simulink model "plasma_load"  (R2026a)
settings: Solver=FixedStepDiscrete  StartTime=0  StopTime=30  FixedStep=1e-5
libraries: ee_lib x17, nesl_utility x13, fl_lib x9
settings Model: ModifiedByFormat=GKC3-Simulink contributors  Creator=GKC3-Simulink contributors  LastModifiedBy=GKC3-Simulink contributors
settings DataIOCC: FinalStateName=xHalf  InitialState=xHalf

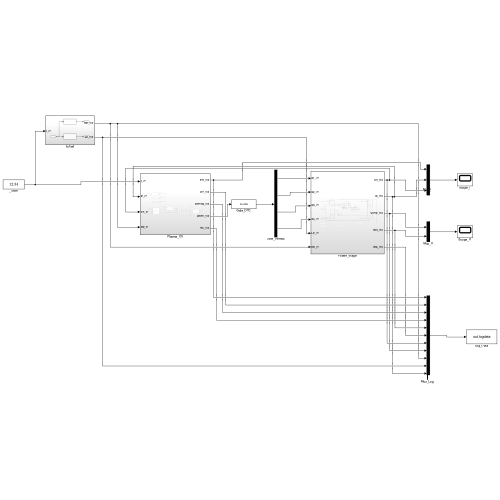
[thumbnail: Simulink's stored preview of the top-level diagram]
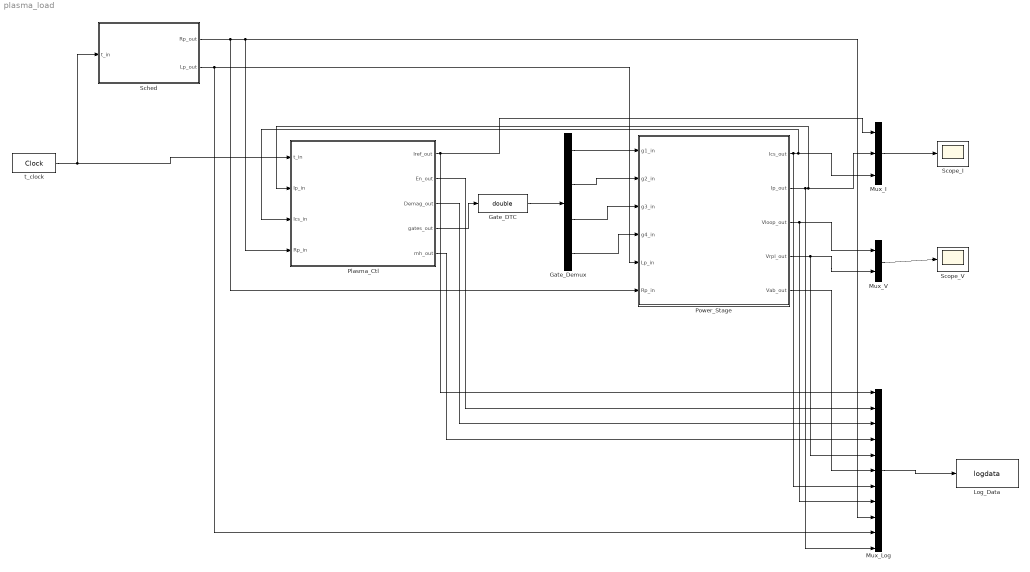
== system plasma_load ==
  Gate_DTC : DataTypeConversion  OutDataTypeStr=double  SaturateOnIntegerOverflow=off  RndMeth=Floor
  Gate_Demux : Demux
  Log_Data : ToWorkspace  VariableName=logdata  SaveFormat=Timeseries  SampleTime=1e-5
  Mux_I : Mux  Inputs=3
  Mux_Log : Mux  Inputs=11
  Mux_V : Mux  Inputs=2
  Plasma_Ctl : Subsystem
  Power_Stage : Subsystem
  Sched : Subsystem
  Scope_I : Scope
  Scope_V : Scope
  t_clock : DigitalClock  SampleTime=1e-5
  wires:
  Plasma_Ctl/4(gates_out) -> Gate_DTC/1
  Gate_DTC/1 -> Gate_Demux/1
  Gate_Demux/1 -> Power_Stage/1(g1_in)
  Gate_Demux/2 -> Power_Stage/2(g2_in)
  Gate_Demux/3 -> Power_Stage/3(g3_in)
  Gate_Demux/4 -> Power_Stage/4(g4_in)
  Mux_V/1 -> Scope_V/1
  t_clock/1 -> Sched/1(t_in), Plasma_Ctl/1(t_in)
  Sched/1(Rp_out) -> Plasma_Ctl/4(Rp_in), Mux_Log/9, Power_Stage/6(Rp_in)
  Sched/2(Lp_out) -> Power_Stage/5(Lp_in), Mux_Log/10
  Power_Stage/1(Ics_out) -> Mux_I/3, Plasma_Ctl/3(Ics_in), Mux_Log/7
  Power_Stage/2(Ip_out) -> Mux_I/2, Plasma_Ctl/2(Ip_in), Mux_Log/11
  Plasma_Ctl/1(Iref_out) -> Mux_Log/1, Mux_I/1
  Power_Stage/3(Vloop_out) -> Mux_V/1, Mux_Log/8
  Power_Stage/4(Vrpl_out) -> Mux_V/2, Mux_Log/5
  Plasma_Ctl/2(En_out) -> Mux_Log/2
  Plasma_Ctl/3(Demag_out) -> Mux_Log/3
  Plasma_Ctl/5(mh_out) -> Mux_Log/4
  Power_Stage/5(Vab_out) -> Mux_Log/6
  Mux_Log/1 -> Log_Data/1
  Mux_I/1 -> Scope_I/1

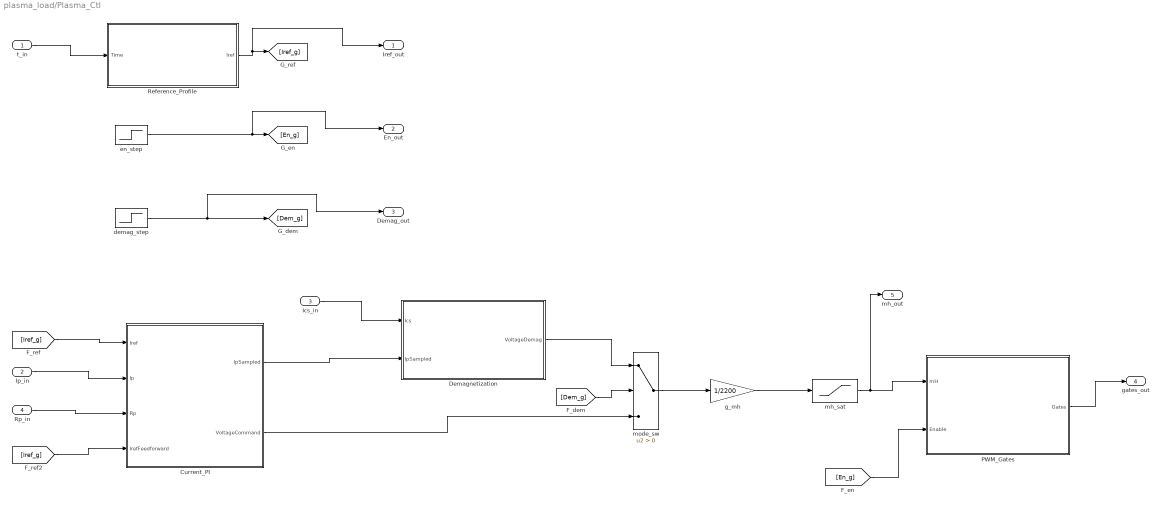
== system plasma_load/Plasma_Ctl ==
  t_in : Inport
  Ip_in : Inport  Port=2
  Ics_in : Inport  Port=3
  Rp_in : Inport  Port=4
  Current_PI : Subsystem
  Demagnetization : Subsystem
  PWM_Gates : Subsystem
  Reference_Profile : Subsystem
  demag_step : Step  Time=12.3  SampleTime=0
  en_step : Step  Time=0.6  SampleTime=0
  g_mh : Gain  Gain=1/2200
  mh_sat : Saturate  UpperLimit=0.95  LowerLimit=-0.95
  mode_sw : Switch  Criteria=u2 > Threshold  SaturateOnIntegerOverflow=off  InputSameDT=off
  Iref_out : Outport
  En_out : Outport  Port=2
  Demag_out : Outport  Port=3
  gates_out : Outport  Port=4
  mh_out : Outport  Port=5
  wires:
  mode_sw/1 -> g_mh/1
  [Dem_g] -> mode_sw/2
  demag_step/1 -> [Dem_g], Demag_out/1
  en_step/1 -> [En_g], En_out/1
  PWM_Gates/1(Gates) -> gates_out/1
  [En_g] -> PWM_Gates/2(Enable)
  Demagnetization/1(VoltageDemag) -> mode_sw/1
  Current_PI/1(IpSampled) -> Demagnetization/2(IpSampled)
  Ics_in/1 -> Demagnetization/1(Ics)
  Current_PI/2(VoltageCommand) -> mode_sw/3
  [Iref_g] -> Current_PI/4(IrefFeedforward)
  Rp_in/1 -> Current_PI/3(Rp)
  Ip_in/1 -> Current_PI/2(Ip)
  [Iref_g] -> Current_PI/1(Iref)
  t_in/1 -> Reference_Profile/1(Time)
  Reference_Profile/1(Iref) -> Iref_out/1, [Iref_g]
  g_mh/1 -> mh_sat/1
  mh_sat/1 -> PWM_Gates/1(mH), mh_out/1

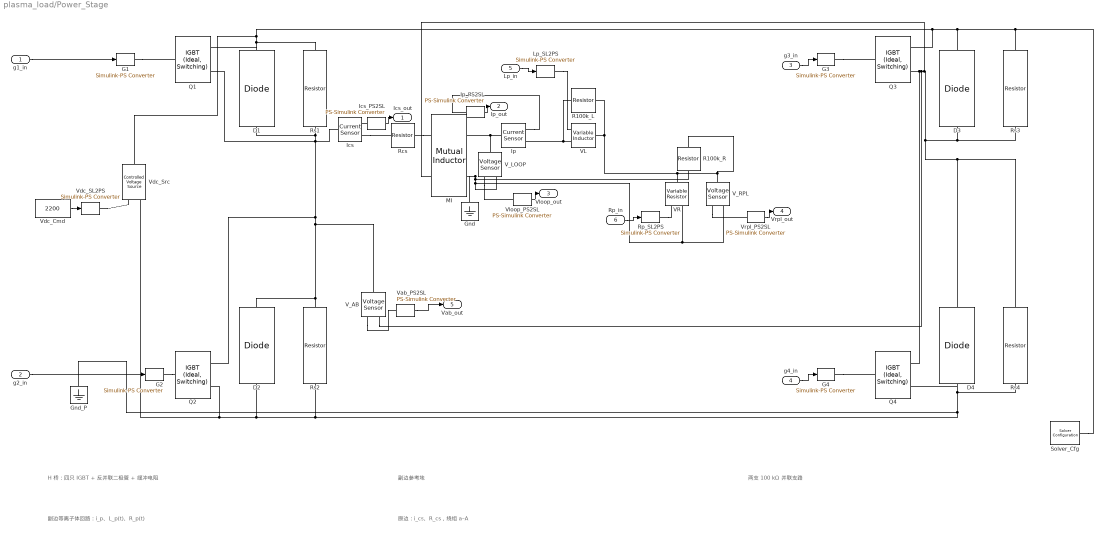
== system plasma_load/Power_Stage ==
  note: 原边：i_cs、R_cs，绕组 a–A
  note: 副边等离子体回路：i_p、L_p(t)、R_p(t)
  note: 两支 100 kΩ 并联支路
  note: 副边参考地
  note: H 桥：四只 IGBT + 反并联二极管 + 缓冲电阻
  g1_in : Inport
  g2_in : Inport  Port=2
  g3_in : Inport  Port=3
  g4_in : Inport  Port=4
  Lp_in : Inport  Port=5
  Rp_in : Inport  Port=6
  D{1..4} (4 alike) : ee_lib/Semiconductors & Converters/Diode  ModelType=ee.enum.diode.modelType.pwl  TableType=ee.enum.diode.tableType.IfMat  IfMat=[.07, .12, .19, 1.75, 4.24, 7.32, 11.2; .16, .3, .72, 2.14, 5.02, 8.35, 13.12] A  VfMat=[.9, 1.15, 1.25, 1.5, 1.75, 2.17, 2.6, 2.85; .58, .68, .75, 1.1, 1.38, 1.77, 2.27, 2.7] V  TjVec=[25, 125] degC  VfVec=[.5, .7, .9, 1.3, 1.7, 2.1, 2.5] V  IfVec=[.1, .2, .5, 1, 2, 4, 7, 10] A  IrMat=[1e-06, 2e-06, 5e-06, 1e-05, 2.5e-05, 5e-05, .0001; 2e-06, 5e-06, 1e-05, 4e-05, 8e-05, .0002, .0005] A  VrMat=[10, 100, 200, 250, 300, 325, 350; 10, 70, 160, 220, 270, 300, 320] V  VrVec=[10, 20, 40, 50, 70, 80, 100] V  IrVec=[1e-06, 2e-06, 5e-06, 1e-05, 2e-05, 5e-05, .0001] A  Vf=2 V  Ron=20e-6 Ohm  Goff=1e-8 S  prmExp=ee.enum.diode.expParam.useTwo  I12=[.0137, .545] A  V12=[.6, .7] V  RS=0 Ohm  Tmeas=298.15 K  IS=1e-12 A  ec=1  I1=0.0137 A  V1=0.6 V  N_series=1  N_parallel=1  ZenerEnable=false  Rz=0.3 Ohm  BV=30 V  C_param=ee.enum.diode.capParam.fixed  CJ=0 pF  CJ0=5 pF  Vvec=[.1, 10, 100] V  Cvec=[3.5, 1, .4] pF  VJ=1 V  Mgrad=0.5  FC=0.5  Q_param=ee.enum.diode.recoveryParam.off  iRM=-7.15 A  iF=4 A  didt=-750 A/us  trr_factor=3  trr=115 ns  Qrr=150 nA*s  Vr=-600 V  Ls=150 nH  Erec=0.03 J  TT=50 ns  tau=100 ns  T_param=ee.enum.diode.temperatureParam.off  Tdevice=298.15 K  I1_T2=0.245 A  V1_T2=0.5 V  IS_T2=1.25e-7 A  Tmeas2=125 degC  XTI_param=ee.enum.diode.xtiParam.pn  XTI=3  EG_param=ee.enum.diode.egapParam.material_si  EG=1.11 eV  dBVdT=0 V/K  enable_fault_input=simscape.enum.onoff.off  i_specify=off  i_priority=None  i=0 A  i_nominal_specify=off  i_nominal_value=1  i_nominal_unit=A  v_specify=off  v_priority=None  v=0 V  v_nominal_specify=off  v_nominal_value=1  v_nominal_unit=V  v_capacitor_specify=off  v_capacitor_priority=None  v_capacitor=0 V  v_capacitor_nominal_specify=off  v_capacitor_nominal_value=1  v_capacitor_nominal_unit=V  Qj_specify=off  Qj_priority=High  Qj=0 C  Qj_nominal_specify=off  Qj_nominal_value=1  Qj_nominal_unit=C  i_diode_specify=off  i_diode_priority=None  i_diode=0 A  i_diode_nominal_specify=off  i_diode_nominal_value=1  i_diode_nominal_unit=A  v_diode_specify=off  v_diode_priority=None  v_diode=0 V  v_diode_nominal_specify=off  v_diode_nominal_value=1  v_diode_nominal_unit=V  i_capacitor_specify=off  i_capacitor_priority=None  i_capacitor=0 A  i_capacitor_nominal_specify=off  i_capacitor_nominal_value=1  i_capacitor_nominal_unit=A  fidelity_level=ee.enum.diode.fidelity.includeChargeDyn  rec_loss_model=ee.enum.diode.reverseRecoveryModelTabulateUpTo3D.fixed  ErecVal=0 J  scaleWithIandV=true  ErecMat=zeros(2, 3) J  ErecMat3D=zeros(2, 3, 2) J  TjrecVec=[298.15, 398.15] K  IfrecVec=[.1, 1, 10] A  IrecVal=10 A  VrecVal=10 V  VrecVec=[0, 100] V  tFilter=1 / 1000 / 100 s  thermal_network_parameterization=ee.enum.thermalNetworkTopology.junctionCase  Rth=[0, 10] K/W  Rth_Cauer=[1, 3, 10] K/W  Rth_Foster=[.08, .14, .22, .16] K/W  thermal_mass_parameterization=ee.enum.thermalNetwork.timeconstant  thermal_mass=[0, 1] J/K  thermal_mass_Cauer=[.1, .3, 1] J/K  thermal_mass_Foster=[.001, .005, .05, .5] J/K  thermal_time_constant=[0, 10] s  thermal_time_constant_Cauer=[1, 3, 10] s  thermal_time_constant_Foster=[7e-05, .0007, .01, .08] s  thermal_mass_initial_temperatures=[25, 25] degC  thermal_mass_initial_temperatures_Cauer=[25, 25, 25] degC  junction_thermal_mass=0.01 J/K  Tvec_initial_Foster=[25, 25, 25, 25] degC  no_thermal_network=0  junction_temperature_specify=off  junction_temperature_priority=None  junction_temperature=25 degC  junction_temperature_nominal_specify=off  junction_temperature_nominal_value=1  junction_temperature_nominal_unit=degC
  G{1..4} (4 alike) : nesl_utility/Simulink-PS Converter  PhysicalDomain=network_engine_domain  SubClassName=ps_input  LeftPortType=input  RightPortType=output  PseudoPeriodic=off  Frequencies=[]  NoiseDistribution=none  NoiseParameters=[]  Unit=V  AffineConversion=off  FilteringAndDerivatives=zero  SimscapeFilterOrder=1  InputFilterTimeConstant=0.001  UdotUserProvided=0
  Gnd : fl_lib/Electrical/Electrical Elements/Electrical Reference
  Gnd_P : fl_lib/Electrical/Electrical Elements/Electrical Reference
  Ics : fl_lib/Electrical/Electrical Sensors/Current Sensor
  Ics_PS2SL : nesl_utility/PS-Simulink Converter  PhysicalDomain=network_engine_domain  SubClassName=ps_output  LeftPortType=input  RightPortType=output  PseudoPeriodic=off  Frequencies=[]  VectorFormat=inherit  Unit=A  AffineConversion=off
  Ip : fl_lib/Electrical/Electrical Sensors/Current Sensor
  Ip_PS2SL : nesl_utility/PS-Simulink Converter  PhysicalDomain=network_engine_domain  SubClassName=ps_output  LeftPortType=input  RightPortType=output  PseudoPeriodic=off  Frequencies=[]  VectorFormat=inherit  Unit=A  AffineConversion=off
  Lp_SL2PS : nesl_utility/Simulink-PS Converter  PhysicalDomain=network_engine_domain  SubClassName=ps_input  LeftPortType=input  RightPortType=output  PseudoPeriodic=off  Frequencies=[]  NoiseDistribution=none  NoiseParameters=[]  Unit=H  AffineConversion=off  FilteringAndDerivatives=provide  SimscapeFilterOrder=1  InputFilterTimeConstant=0.001  UdotUserProvided=0
  MI : ee_lib/Passive/Transformers/Mutual Inductor  L1=1 H  L2=1 H  k=0.99999  L_tol=20  enable_L1_tol=ee.enum.toleranceApplication.none  L1_tol_distribution=ee.enum.toleranceDistribution.uniform  L1_nSigma=4  enable_L2_tol=ee.enum.toleranceApplication.none  L2_tol_distribution=ee.enum.toleranceDistribution.uniform  L2_nSigma=4  r=[1e-9, 1e-9] Ohm  g=[1e-9, 1e-9] 1/Ohm  enable_operating_limits=ee.enum.enable.no  operating_limit_action=ee.enum.passive.reportOpLim.warn  max_working_current=1 A  power_rating=1 W  iL1_specify=off  iL1_priority=High  iL1=0 A  iL1_nominal_specify=off  iL1_nominal_value=1  iL1_nominal_unit=A  iL2_specify=off  iL2_priority=High  iL2=0 A  iL2_nominal_specify=off  iL2_nominal_value=1  iL2_nominal_unit=A
  Q{1..4} (4 alike) : ee_lib/Semiconductors & Converters/IGBT (Ideal, Switching)  port_option=ee.enum.controlport.ps  Vf=2 V  Ron=20e-6 Ohm  Goff=1e-8 1/Ohm  Vth=0.5 V  diode_param=ee.enum.semiconductors.protectionDiode.external  diode_Vf=0.8 V  diode_Ron=0.001 Ohm  diode_Goff=1e-5 1/Ohm  diode_C=50e-9 F  diode_iRM=-235 A  diode_iF=300 A  diode_idot=-50 A/us  diode_trr_param=ee.enum.converters.diodeReverseParam.trr_factor  diode_trr_factor=3  diode_trr=15 us  diode_Qrr=1500 s*uA  ice_specify=off  ice_priority=None  ice=0 A  ice_nominal_specify=off  ice_nominal_value=1  ice_nominal_unit=A  vce_specify=off  vce_priority=None  vce=0 V  vce_nominal_specify=off  vce_nominal_value=1  vce_nominal_unit=V  vge_specify=off  vge_priority=None  vge=0 V  vge_nominal_specify=off  vge_nominal_value=1  vge_nominal_unit=V  thermal_loss_option=ee.enum.converters.thermalLossOption.constantvalues  Von_data=[0, .1, .6, .8, 1, 1.3, 1.6, 2, 2.4; 0, .1, .7, 1, 1.2, 1.5, 1.9, 2.4, 2.8] V  Tj=[298.15, 398.15] K  Iout_data=[0, .1, 1, 5, 10, 20, 40, 70, 100] A  tabulateWithVce=false  Eon_data=[0, .0024, .024, .12, .2, .48, 1.04, 2.16, 3.24; 0, .003, .03, .15, .25, .6, 1.3, 2.7, 4.05] * 1e-3 J  Eoff_data=[0, .0007, .0066, .033, .066, .17, .33, .83, 1.5; 0, .001, .01, .05, .1, .25, .5, 1.2, 2.2] * 1e-3 J  Eon_data_3D=[zeros(2, 9, 3)] J  Eoff_data_3D=[zeros(2, 9, 3)] J  Tj_loss=[298.15, 398.15] K  Iout_data_loss=[0, .1, 1, 5, 10, 20, 40, 70, 100] A  Vce_loss=[0, 150, 300] V  Eon_scalar=22.86e-3 J  Eoff_scalar=17.14e-3 J  Voff=300 V  Iout_scalar=600 A  useCurrentFromPreviousCycle=false  useVoltageFromPreviousCycle=false  diodeModelType=ee.enum.converters.diodeModelType.pwl  diodeTableType=ee.enum.diode.tableType.IfMat  diode_ReverseIVType=ee.enum.diode.diodeReverseIV.constant  diode_IfMat=[.07, .12, .19, 1.75, 4.24, 7.32, 11.2; .16, .3, .72, 2.14, 4.02, 6.35, 9.12] A  diode_VfMat=[.9, 1.15, 1.25, 1.5, 1.75, 2.17, 2.6, 2.85; .58, .68, .75, 1.1, 1.38, 1.77, 2.27, 2.7] V  diode_TjVec=[25, 125] degC  diode_VfVec=[.5, .7, .9, 1.3, 1.7, 2.1, 2.5] V  diode_IfVec=[.1, .2, .5, 1, 2, 4, 7, 10] A  diode_IrMat=[1e-06, 2e-06, 5e-06, 1e-05, 2.5e-05, 5e-05, .0001; 2e-06, 5e-06, 1e-05, 4e-05, 8e-05, .0002, .0005] A  diode_VrMat=[10, 100, 200, 250, 300, 325, 350; 10, 70, 160, 220, 270, 300, 320] V  diode_VrVec=[10, 20, 40, 50, 70, 80, 100] V  diode_IrVec=[1e-06, 2e-06, 5e-06, 1e-05, 2e-05, 5e-05, .0001] A  diode_Vr=-600 V  diode_Ls=150 nH  diode_Erec=0.03 J  diode_rec_loss_model=ee.enum.diode.reverseRecoveryModelTabulateUpTo3D.fixed  diode_ErecVal=0 J  diode_scaleWithIandV=true  diode_ErecMat=zeros(2, 3) J  diodeErecMat3D=zeros(2, 3, 2) J  diode_TjrecVec=[298.15, 398.15] K  diode_IfrecVec=[.1, 1, 10] A  diodeVrecVec=[0, 100] V  diode_IrecVal=10 A  diode_VrecVal=10 V  diode_tFilter=1 / 1000 / 100 s  separateThermalPortForDiode=false  thermal_network_parameterization=ee.enum.thermalNetworkTopology.external  Rth=[.08, .5] K/W  Rth_Cauer=[.08, .1, .5] K/W  Rth_Foster=[.08, .14, .22, .16] K/W  thermal_mass_parameterization=ee.enum.thermalNetwork.timeconstant  thermal_mass=[.01, .5] J/K  thermal_mass_Cauer=[.01, .1, .5] J/K  thermal_mass_Foster=[.001, .005, .05, .5] J/K  thermal_time_constant=[.001, .2] s  thermal_time_constant_Cauer=[.001, .1, .2] s  thermal_time_constant_Foster=[7e-05, .0007, .01, .08] s  thermal_mass_initial_temperatures=[25, 25] degC  thermal_mass_initial_temperatures_Cauer=[25, 25, 25] degC  junction_thermal_mass=0.01 J/K  Tvec_initial_Foster=[25, 25, 25, 25] degC  RthDiode=[.03, .2] K/W  RthCauerDiode=[.03, .1, .2] K/W  RthFosterDiode=[.03, .2] K/W  thermalMassDiode=[3, 25] J/K  thermalMassCauerDiode=[3, 10, 25] J/K  thermalMassFosterDiode=[33, 50] J/K  thermalTauDiode=[.1, 5] s  thermalTauCauerDiode=[.1, 1, 5] s  thermalTauFosterDiode=[1, 10] s  thermalMassInitTempDiode=[25, 25] degC  thermalMassInitTempCauerDiode=[25, 25, 25] degC  junctionthermalMassDiode=0.1 J/K  TVecInitialFosterDiode=[25, 25, 25, 25] degC  no_thermal_network=ee.enum.enable.no  IGBT_junction_temperature_specify=off  IGBT_junction_temperature_priority=None  IGBT_junction_temperature=25 degC  IGBT_junction_temperature_nominal_specify=off  IGBT_junction_temperature_nominal_value=1  IGBT_junction_temperature_nominal_unit=degC  diode_junction_temperature_specify=off  diode_junction_temperature_priority=None  diode_junction_temperature=25 degC  diode_junction_temperature_nominal_specify=off  diode_junction_temperature_nominal_value=1  diode_junction_temperature_nominal_unit=degC  Qj_specify=off  Qj_priority=None  Qj=0 W  Qj_nominal_specify=off  Qj_nominal_value=1  Qj_nominal_unit=W  accumulatedSwitchingLosses_specify=off  accumulatedSwitchingLosses_priority=None  accumulatedSwitchingLosses=0 J
  R100k_L : ee_lib/Passive/Resistor  R=1e5 Ohm  enable_R_tol=ee.enum.toleranceApplication.none  R_tol=5  tol_distribution=ee.enum.toleranceDistribution.uniform  nSigma=4  enable_operating_limits=ee.enum.enable.no  operating_limit_action=ee.enum.passive.reportOpLim.warn  power_rating=1 W  max_working_voltage=100 V  noise_mode=ee.enum.sources.noise.Disabled  Tdevice=25 degC  sample_time=1e-3 s  repeatability=ee.enum.ic.repeatability.notRepeatable  user_seed=0  auto_seed=2193747164  power_derating_T1=70 degC  power_derating_T2=155 degC  operating_temperature_range_vec=[-50, 150] degC  alpha=3.93e-3 1/K  Tmeas=25 degC  thermal_mass=100 J/K  temperature_specify=off  temperature_priority=High  temperature=298.15 K  temperature_nominal_specify=off  temperature_nominal_value=1  temperature_nominal_unit=K
  R100k_R : ee_lib/Passive/Resistor  R=1e5 Ohm  enable_R_tol=ee.enum.toleranceApplication.none  R_tol=5  tol_distribution=ee.enum.toleranceDistribution.uniform  nSigma=4  enable_operating_limits=ee.enum.enable.no  operating_limit_action=ee.enum.passive.reportOpLim.warn  power_rating=1 W  max_working_voltage=100 V  noise_mode=ee.enum.sources.noise.Disabled  Tdevice=25 degC  sample_time=1e-3 s  repeatability=ee.enum.ic.repeatability.notRepeatable  user_seed=0  auto_seed=3511684267  power_derating_T1=70 degC  power_derating_T2=155 degC  operating_temperature_range_vec=[-50, 150] degC  alpha=3.93e-3 1/K  Tmeas=25 degC  thermal_mass=100 J/K  temperature_specify=off  temperature_priority=High  temperature=298.15 K  temperature_nominal_specify=off  temperature_nominal_value=1  temperature_nominal_unit=K
  Rcs : ee_lib/Passive/Resistor  R=20e-6 Ohm  enable_R_tol=ee.enum.toleranceApplication.none  R_tol=5  tol_distribution=ee.enum.toleranceDistribution.uniform  nSigma=4  enable_operating_limits=ee.enum.enable.no  operating_limit_action=ee.enum.passive.reportOpLim.warn  power_rating=1 W  max_working_voltage=100 V  noise_mode=ee.enum.sources.noise.Disabled  Tdevice=25 degC  sample_time=1e-3 s  repeatability=ee.enum.ic.repeatability.notRepeatable  user_seed=0  auto_seed=2184028045  power_derating_T1=70 degC  power_derating_T2=155 degC  operating_temperature_range_vec=[-50, 150] degC  alpha=3.93e-3 1/K  Tmeas=25 degC  thermal_mass=100 J/K  temperature_specify=off  temperature_priority=High  temperature=298.15 K  temperature_nominal_specify=off  temperature_nominal_value=1  temperature_nominal_unit=K
  Rp_SL2PS : nesl_utility/Simulink-PS Converter  PhysicalDomain=network_engine_domain  SubClassName=ps_input  LeftPortType=input  RightPortType=output  PseudoPeriodic=off  Frequencies=[]  NoiseDistribution=none  NoiseParameters=[]  Unit=Ohm  AffineConversion=off  FilteringAndDerivatives=provide  SimscapeFilterOrder=1  InputFilterTimeConstant=0.001  UdotUserProvided=0
  Rs1 : ee_lib/Passive/Resistor  R=1e7 Ohm  enable_R_tol=ee.enum.toleranceApplication.none  R_tol=5  tol_distribution=ee.enum.toleranceDistribution.uniform  nSigma=4  enable_operating_limits=ee.enum.enable.no  operating_limit_action=ee.enum.passive.reportOpLim.warn  power_rating=1 W  max_working_voltage=100 V  noise_mode=ee.enum.sources.noise.Disabled  Tdevice=25 degC  sample_time=1e-3 s  repeatability=ee.enum.ic.repeatability.notRepeatable  user_seed=0  auto_seed=2090754141  power_derating_T1=70 degC  power_derating_T2=155 degC  operating_temperature_range_vec=[-50, 150] degC  alpha=3.93e-3 1/K  Tmeas=25 degC  thermal_mass=100 J/K  temperature_specify=off  temperature_priority=High  temperature=298.15 K  temperature_nominal_specify=off  temperature_nominal_value=1  temperature_nominal_unit=K
  Rs2 : ee_lib/Passive/Resistor  R=1e7 Ohm  enable_R_tol=ee.enum.toleranceApplication.none  R_tol=5  tol_distribution=ee.enum.toleranceDistribution.uniform  nSigma=4  enable_operating_limits=ee.enum.enable.no  operating_limit_action=ee.enum.passive.reportOpLim.warn  power_rating=1 W  max_working_voltage=100 V  noise_mode=ee.enum.sources.noise.Disabled  Tdevice=25 degC  sample_time=1e-3 s  repeatability=ee.enum.ic.repeatability.notRepeatable  user_seed=0  auto_seed=1871998384  power_derating_T1=70 degC  power_derating_T2=155 degC  operating_temperature_range_vec=[-50, 150] degC  alpha=3.93e-3 1/K  Tmeas=25 degC  thermal_mass=100 J/K  temperature_specify=off  temperature_priority=High  temperature=298.15 K  temperature_nominal_specify=off  temperature_nominal_value=1  temperature_nominal_unit=K
  Rs3 : ee_lib/Passive/Resistor  R=1e7 Ohm  enable_R_tol=ee.enum.toleranceApplication.none  R_tol=5  tol_distribution=ee.enum.toleranceDistribution.uniform  nSigma=4  enable_operating_limits=ee.enum.enable.no  operating_limit_action=ee.enum.passive.reportOpLim.warn  power_rating=1 W  max_working_voltage=100 V  noise_mode=ee.enum.sources.noise.Disabled  Tdevice=25 degC  sample_time=1e-3 s  repeatability=ee.enum.ic.repeatability.notRepeatable  user_seed=0  auto_seed=1918921592  power_derating_T1=70 degC  power_derating_T2=155 degC  operating_temperature_range_vec=[-50, 150] degC  alpha=3.93e-3 1/K  Tmeas=25 degC  thermal_mass=100 J/K  temperature_specify=off  temperature_priority=High  temperature=298.15 K  temperature_nominal_specify=off  temperature_nominal_value=1  temperature_nominal_unit=K
  Rs4 : ee_lib/Passive/Resistor  R=1e7 Ohm  enable_R_tol=ee.enum.toleranceApplication.none  R_tol=5  tol_distribution=ee.enum.toleranceDistribution.uniform  nSigma=4  enable_operating_limits=ee.enum.enable.no  operating_limit_action=ee.enum.passive.reportOpLim.warn  power_rating=1 W  max_working_voltage=100 V  noise_mode=ee.enum.sources.noise.Disabled  Tdevice=25 degC  sample_time=1e-3 s  repeatability=ee.enum.ic.repeatability.notRepeatable  user_seed=0  auto_seed=1315760964  power_derating_T1=70 degC  power_derating_T2=155 degC  operating_temperature_range_vec=[-50, 150] degC  alpha=3.93e-3 1/K  Tmeas=25 degC  thermal_mass=100 J/K  temperature_specify=off  temperature_priority=High  temperature=298.15 K  temperature_nominal_specify=off  temperature_nominal_value=1  temperature_nominal_unit=K
  Solver_Cfg : nesl_utility/Solver Configuration  PhysicalDomain=network_engine_domain  SubClassName=solver  LeftPortType=input  RightPortType=generic  Tones=[]  Harmonics=[]  SimulateNoise=off  Profile=off  UseLocalSampling=off  EnableSwitchedLinearOptims=on  FrequencyDomain=off  UseCCode=off  RelTol=0.001  AbsTol=0.001  MinStep=1e-09  ToWorkspace=off  RevertToSquareIcSolve=off  NumHomotopyIterations=100  PhasorMode=off  PhasorModeNumHarmonics=1  ConsistencySolver=NEWTON_XTOL_AFTER_FTOL  CanonicalOrdering=CANONICAL  OptimizeIntermediates=OPTIMIZED  IndexReductionMethod=DerivativeReplacement  DoDC=off  ResidualTolerance=1e-09  ConsistencyTolSource=GLOBAL  ConsistencyAbsTol=0.001  ConsistencyRelTol=0.001  ConsistencyTolFactor=0.001  UseLocalSolver=on  LocalSolverChoice=NE_BACKWARD_EULER_ADVANCER  ResolveIndetEquations=on  FunctionEvalNumThread=1  LocalSolverSampleTime=1e-5  DoFixedCost=on  MaxNonlinIter=3  MaxModeIter=2  ComputeImpulses=off  ImpulseIterations=2  LinearAlgebra=auto  LinearAlgebraNumThread=0  EquationFormulation=NE_TIME_EF  DelaysMemoryBudget=1024  AutomaticFiltering=on  FilteringTimeConstant=0.001  PartitionStorageMethod=AS_NEEDED  PartitionMemoryBudget=1024  PartitionMethod=ROBUST  MultibodyUseLocalSolver=off  MultibodyLocalSolverChoice=ODE1  MultibodyLocalSolverSampleTime=0.001
  VL : ee_lib/Passive/Variable Inductor  prm=1  Lmin=1e-6 H  g=1e-9 1/Ohm  i0=0 A  phi0=0 Wb
  VR : fl_lib/Electrical/Electrical Elements/Variable Resistor  Rmin=1e-5 Ohm  thermalEnable=false  thermal_mass=1 J/K  i_specify=off  i_priority=None  i=0 A  i_nominal_specify=off  i_nominal_value=1  i_nominal_unit=A  v_specify=off  v_priority=None  v=0 V  v_nominal_specify=off  v_nominal_value=1  v_nominal_unit=V  T_specify=off  T_priority=None  T=300 K  T_nominal_specify=off  T_nominal_value=1  T_nominal_unit=K
  V_AB : fl_lib/Electrical/Electrical Sensors/Voltage Sensor
  V_LOOP : fl_lib/Electrical/Electrical Sensors/Voltage Sensor
  V_RPL : fl_lib/Electrical/Electrical Sensors/Voltage Sensor
  Vab_PS2SL : nesl_utility/PS-Simulink Converter  PhysicalDomain=network_engine_domain  SubClassName=ps_output  LeftPortType=input  RightPortType=output  PseudoPeriodic=off  Frequencies=[]  VectorFormat=inherit  Unit=V  AffineConversion=off
  Vdc_Cmd : Constant  Value=2200
  Vdc_SL2PS : nesl_utility/Simulink-PS Converter  PhysicalDomain=network_engine_domain  SubClassName=ps_input  LeftPortType=input  RightPortType=output  PseudoPeriodic=off  Frequencies=[]  NoiseDistribution=none  NoiseParameters=[]  Unit=V  AffineConversion=off  FilteringAndDerivatives=zero  SimscapeFilterOrder=1  InputFilterTimeConstant=0.001  UdotUserProvided=0
  Vdc_Src : fl_lib/Electrical/Electrical Sources/Controlled Voltage Source
  Vloop_PS2SL : nesl_utility/PS-Simulink Converter  PhysicalDomain=network_engine_domain  SubClassName=ps_output  LeftPortType=input  RightPortType=output  PseudoPeriodic=off  Frequencies=[]  VectorFormat=inherit  Unit=V  AffineConversion=off
  Vrpl_PS2SL : nesl_utility/PS-Simulink Converter  PhysicalDomain=network_engine_domain  SubClassName=ps_output  LeftPortType=input  RightPortType=output  PseudoPeriodic=off  Frequencies=[]  VectorFormat=inherit  Unit=V  AffineConversion=off
  Ics_out : Outport
  Ip_out : Outport  Port=2
  Vloop_out : Outport  Port=3
  Vrpl_out : Outport  Port=4
  Vab_out : Outport  Port=5
  wires:
  Vab_PS2SL/1 -> Vab_out/1
  Vrpl_PS2SL/1 -> Vrpl_out/1
  Vloop_PS2SL/1 -> Vloop_out/1
  Ip_PS2SL/1 -> Ip_out/1
  Ics_PS2SL/1 -> Ics_out/1
  Rp_in/1 -> Rp_SL2PS/1
  Lp_in/1 -> Lp_SL2PS/1
  g4_in/1 -> G4/1
  g3_in/1 -> G3/1
  g2_in/1 -> G2/1
  g1_in/1 -> G1/1
  Vdc_Cmd/1 -> Vdc_SL2PS/1
  connections:
  Vdc_SL2PS/RConn1 -- Vdc_Src/RConn1
  Q3/RConn1 -- Solver_Cfg/RConn1 -- Rs3/RConn1 -- D3/RConn1 -- Rs1/RConn1 -- D1/RConn1 -- Q1/RConn1 -- Vdc_Src/LConn1
  Vdc_Src/RConn2 -- Q4/RConn2 -- Rs4/LConn1 -- D4/LConn1 -- Gnd_P/LConn1 -- Rs2/LConn1 -- D2/LConn1 -- Q2/RConn2
  D2/RConn1 -- D1/LConn1 -- Rs1/LConn1 -- Ics/LConn1 -- Q1/RConn2 -- Q2/RConn1 -- V_AB/LConn1 -- Rs2/RConn1
  Q4/RConn1 -- Rs4/RConn1 -- D4/RConn1 -- Rs3/LConn1 -- D3/LConn1 -- MI/LConn2 -- V_AB/RConn2 -- Q3/RConn2
  MI/RConn1 -- V_LOOP/LConn1 -- Ip/LConn1
  Ip/RConn2 -- R100k_L/LConn1 -- VL/LConn2
  VR/RConn1 -- R100k_L/RConn1 -- VL/RConn1 -- R100k_R/RConn1 -- V_RPL/LConn1
  VR/LConn2 -- Gnd/LConn1 -- MI/RConn2 -- R100k_R/LConn1 -- V_LOOP/RConn2 -- V_RPL/RConn2
  V_AB/RConn1 -- Vab_PS2SL/LConn1
  V_RPL/RConn1 -- Vrpl_PS2SL/LConn1
  V_LOOP/RConn1 -- Vloop_PS2SL/LConn1
  Ip/RConn1 -- Ip_PS2SL/LConn1
  Ics/RConn1 -- Ics_PS2SL/LConn1
  Rp_SL2PS/RConn1 -- VR/LConn1
  Lp_SL2PS/RConn1 -- VL/LConn1
  Rcs/RConn1 -- MI/LConn1
  Ics/RConn2 -- Rcs/LConn1
  G4/RConn1 -- Q4/LConn1
  G3/RConn1 -- Q3/LConn1
  G2/RConn1 -- Q2/LConn1
  G1/RConn1 -- Q1/LConn1

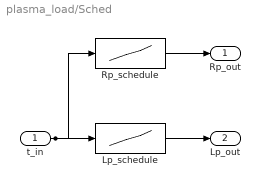
== system plasma_load/Sched ==
  t_in : Inport
  Lp_schedule : Lookup_n-D  NumberOfTableDimensions=1  BreakpointsForDimension1=[0 0.6 1.6 30]  Table=[150e-6 150e-6 100e-6 100e-6]  ExtrapMethod=Clip  InternalRulePriority=Speed  RndMeth=Simplest
  Rp_schedule : Lookup_n-D  NumberOfTableDimensions=1  BreakpointsForDimension1=[0 0.6 1.6 11.6 12.1 12.3 30]  Table=[0.015 0.015 0.01 0.01 0.01 100 100]  ExtrapMethod=Clip  InternalRulePriority=Speed  RndMeth=Simplest
  Rp_out : Outport
  Lp_out : Outport  Port=2
  wires:
  Lp_schedule/1 -> Lp_out/1
  Rp_schedule/1 -> Rp_out/1
  t_in/1 -> Lp_schedule/1, Rp_schedule/1

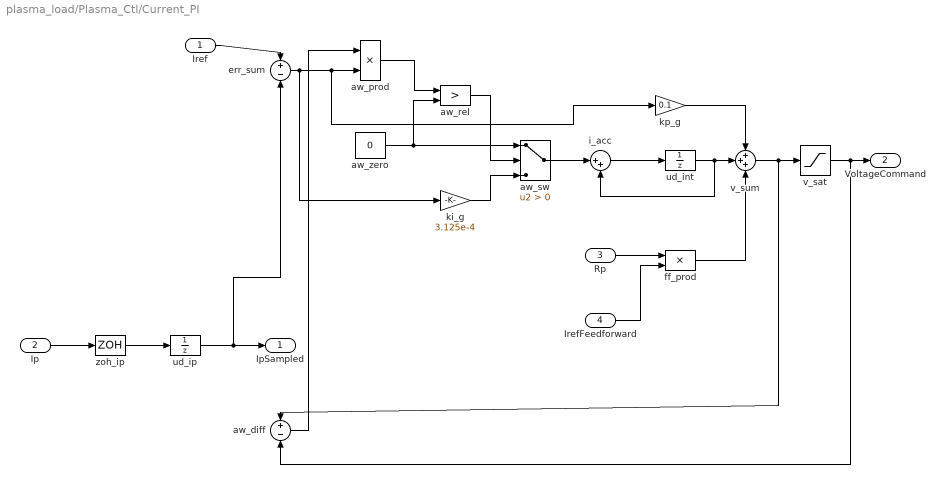
== system plasma_load/Plasma_Ctl/Current_PI ==
  Iref : Inport
  Ip : Inport  Port=2
  Rp : Inport  Port=3
  IrefFeedforward : Inport  Port=4
  aw_diff : Sum  Inputs=+-
  aw_prod : Product
  aw_rel : RelationalOperator  Operator=>  OutDataTypeStr=boolean  RndMeth=Simplest  InputSameDT=off
  aw_sw : Switch  Criteria=u2 > Threshold  SaturateOnIntegerOverflow=off  InputSameDT=off
  aw_zero : Constant  Value=0
  err_sum : Sum  Inputs=+-
  ff_prod : Product
  i_acc : Sum  Inputs=|++
  ki_g : Gain  Gain=3.125e-4
  kp_g : Gain  Gain=0.1
  ud_int : UnitDelay  SampleTime=50e-6
  ud_ip : UnitDelay  SampleTime=50e-6
  v_sat : Saturate  UpperLimit=400  LowerLimit=-400
  v_sum : Sum  Inputs=+++
  zoh_ip : ZeroOrderHold  SampleTime=50e-6
  IpSampled : Outport
  VoltageCommand : Outport  Port=2
  wires:
  aw_prod/1 -> aw_rel/1
  zoh_ip/1 -> ud_ip/1
  aw_diff/1 -> aw_prod/1
  aw_zero/1 -> aw_sw/1, aw_rel/2
  aw_rel/1 -> aw_sw/2
  Iref/1 -> err_sum/1
  ki_g/1 -> aw_sw/3
  v_sat/1 -> aw_diff/2, VoltageCommand/1
  ud_ip/1 -> err_sum/2, IpSampled/1
  i_acc/1 -> ud_int/1
  aw_sw/1 -> i_acc/1
  Rp/1 -> ff_prod/1
  Ip/1 -> zoh_ip/1
  IrefFeedforward/1 -> ff_prod/2
  v_sum/1 -> aw_diff/1, v_sat/1
  kp_g/1 -> v_sum/1
  err_sum/1 -> kp_g/1, aw_prod/2, ki_g/1
  ff_prod/1 -> v_sum/3
  ud_int/1 -> v_sum/2, i_acc/2

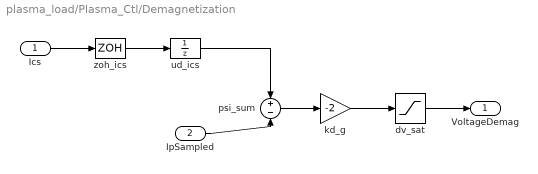
== system plasma_load/Plasma_Ctl/Demagnetization ==
  Ics : Inport
  IpSampled : Inport  Port=2
  dv_sat : Saturate  UpperLimit=400  LowerLimit=-400
  kd_g : Gain  Gain=-2
  psi_sum : Sum  Inputs=+-
  ud_ics : UnitDelay  SampleTime=50e-6
  zoh_ics : ZeroOrderHold  SampleTime=50e-6
  VoltageDemag : Outport
  wires:
  psi_sum/1 -> kd_g/1
  kd_g/1 -> dv_sat/1
  IpSampled/1 -> psi_sum/2
  Ics/1 -> zoh_ics/1
  zoh_ics/1 -> ud_ics/1
  ud_ics/1 -> psi_sum/1
  dv_sat/1 -> VoltageDemag/1

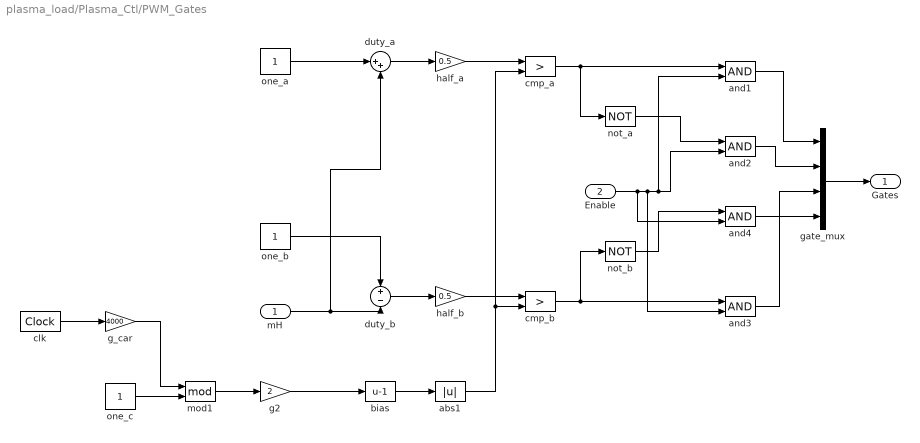
== system plasma_load/Plasma_Ctl/PWM_Gates ==
  mH : Inport
  Enable : Inport  Port=2
  abs1 : Abs  SaturateOnIntegerOverflow=off
  and{1..4} (4 alike) : Logic  IconShape=distinctive  AllPortsSameDT=off  OutDataTypeStr=boolean
  bias : Bias  Bias=-1  SaturateOnIntegerOverflow=off
  clk : DigitalClock  SampleTime=1e-5
  cmp_a : RelationalOperator  Operator=>  OutDataTypeStr=boolean  RndMeth=Simplest  InputSameDT=off
  cmp_b : RelationalOperator  Operator=>  OutDataTypeStr=boolean  RndMeth=Simplest  InputSameDT=off
  duty_a : Sum  Inputs=|++
  duty_b : Sum  Inputs=+-
  g2 : Gain  Gain=2
  g_car : Gain  Gain=4000
  gate_mux : Mux
  half_a : Gain  Gain=0.5
  half_b : Gain  Gain=0.5
  mod1 : Math  Operator=mod
  not_a : Logic  Operator=NOT  IconShape=distinctive  AllPortsSameDT=off  OutDataTypeStr=boolean
  not_b : Logic  Operator=NOT  IconShape=distinctive  AllPortsSameDT=off  OutDataTypeStr=boolean
  one_a : Constant
  one_b : Constant
  one_c : Constant
  Gates : Outport
  wires:
  bias/1 -> abs1/1
  mod1/1 -> g2/1
  clk/1 -> g_car/1
  not_b/1 -> and4/1
  cmp_a/1 -> not_a/1, and1/1
  and2/1 -> gate_mux/2
  gate_mux/1 -> Gates/1
  one_b/1 -> duty_b/1
  abs1/1 -> cmp_a/2, cmp_b/2
  g_car/1 -> mod1/1
  and4/1 -> gate_mux/4
  one_a/1 -> duty_a/1
  and3/1 -> gate_mux/3
  duty_b/1 -> half_b/1
  one_c/1 -> mod1/2
  half_a/1 -> cmp_a/1
  g2/1 -> bias/1
  duty_a/1 -> half_a/1
  and1/1 -> gate_mux/1
  cmp_b/1 -> not_b/1, and3/1
  half_b/1 -> cmp_b/1
  not_a/1 -> and2/1
  mH/1 -> duty_a/2, duty_b/2
  Enable/1 -> and2/2, and1/2, and3/2, and4/2

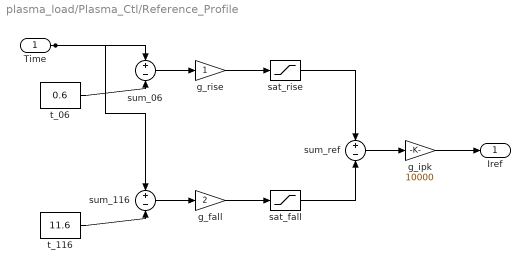
== system plasma_load/Plasma_Ctl/Reference_Profile ==
  Time : Inport
  g_fall : Gain  Gain=2
  g_ipk : Gain  Gain=10000
  g_rise : Gain
  sat_fall : Saturate  UpperLimit=1  LowerLimit=0
  sat_rise : Saturate  UpperLimit=1  LowerLimit=0
  sum_06 : Sum  Inputs=+-
  sum_116 : Sum  Inputs=+-
  sum_ref : Sum  Inputs=+-
  t_06 : Constant  Value=0.6
  t_116 : Constant  Value=11.6
  Iref : Outport
  wires:
  g_fall/1 -> sat_fall/1
  g_rise/1 -> sat_rise/1
  sum_06/1 -> g_rise/1
  g_ipk/1 -> Iref/1
  sat_rise/1 -> sum_ref/1
  sat_fall/1 -> sum_ref/2
  Time/1 -> sum_06/1, sum_116/1
  t_06/1 -> sum_06/2
  sum_ref/1 -> g_ipk/1
  t_116/1 -> sum_116/2
  sum_116/1 -> g_fall/1
